simulink model "S11_telemedicine_simulation"  (R2026a)
settings: Solver=VariableStepAuto  StopTime=600
settings Model: Creator=Aditya  LastModifiedBy=purna

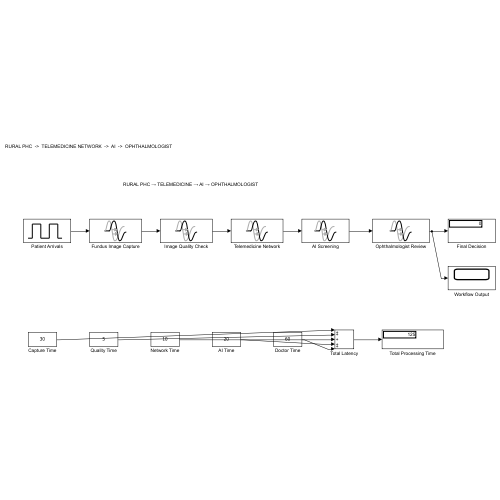
[thumbnail: Simulink's stored preview of the top-level diagram]
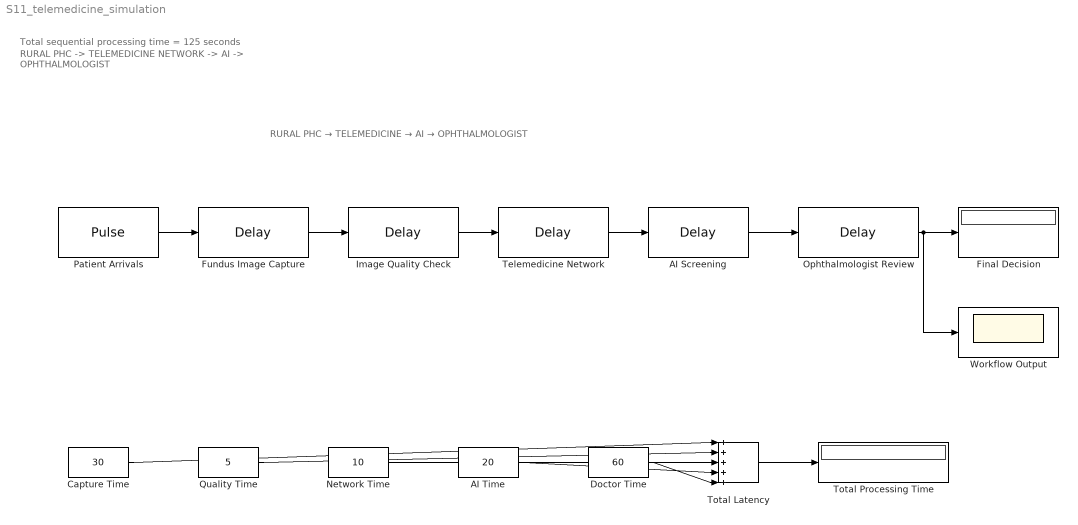
== system S11_telemedicine_simulation ==
  note: RURAL PHC → TELEMEDICINE → AI → OPHTHALMOLOGIST
  note: RURAL PHC -> TELEMEDICINE NETWORK -> AI -> OPHTHALMOLOGIST
  note: Total sequential processing time = 125 seconds
  AI Screening : TransportDelay  DelayTime=20
  AI Time : Constant  Value=20
  Capture Time : Constant  Value=30
  Doctor Time : Constant  Value=60
  Final Decision : Display
  Fundus Image Capture : TransportDelay  DelayTime=30
  Image Quality Check : TransportDelay  DelayTime=5
  Network Time : Constant  Value=10
  Ophthalmologist Review : TransportDelay  DelayTime=60
  Patient Arrivals : DiscretePulseGenerator  PulseType=Time based  Period=60  PulseWidth=10
  Quality Time : Constant  Value=5
  Telemedicine Network : TransportDelay  DelayTime=10
  Total Latency : Sum  Inputs=+++++
  Total Processing Time : Display
  Workflow Output : Scope
      settings: ActiveDisplayYMinimum=-0.38020833333333326  ActiveDisplayYMaximum=0.82928240740740744
  wires:
  Patient Arrivals/1 -> Fundus Image Capture/1
  Fundus Image Capture/1 -> Image Quality Check/1
  Image Quality Check/1 -> Telemedicine Network/1
  Telemedicine Network/1 -> AI Screening/1
  AI Screening/1 -> Ophthalmologist Review/1
  Ophthalmologist Review/1 -> Final Decision/1, Workflow Output/1
  Capture Time/1 -> Total Latency/1
  Quality Time/1 -> Total Latency/2
  Network Time/1 -> Total Latency/3
  AI Time/1 -> Total Latency/4
  Doctor Time/1 -> Total Latency/5
  Total Latency/1 -> Total Processing Time/1
